simulink model "isitici"  (R2026b)
settings: Solver=VariableStepAuto  StopTime=1200  MaxStep=0.1
values from neighbouring files (symbols this model uses):
  Chx = 10000    [init_params.m]
  cpw = 4186    [init_params.m]    (also in test_ch_low.m)
  Crad = 100000    [init_params.m]
  Croom = 2e6    (= 2000000)    [init_params.m]
  dTmax = 30    [init_params.m]
  etanom = 0.975    [init_params.m]
  etax = [30 55 80]    [init_params.m]
  etay = [1.02 0.975 0.975]    [init_params.m]
  hcmode = 1    [init_params.m]    (also in test_hc.m = 2; test_room.m = 2)
  hcx = [-15 -5 5 15 20]    [init_params.m]
  hcy = [75 62 49 36 30]    [init_params.m]    (also in test_hc.m = hcy_backup)
  Kir = 0.002    [init_params.m]
  Kpr = 10    [init_params.m]
  Krad = 35.2    [init_params.m]
  Ktr = 0.5    [init_params.m]
  mdot = 0.25    [init_params.m]
  nmax = 3    [init_params.m]
  nrad = 1.3    [init_params.m]
  Qgasmax = 24600    [init_params.m]
  Qmax = 24000    [init_params.m]
  Qmin = Qmax/turndown    (= 2400)    [init_params.m]
  Tamb = Troomset    (= 21)    [test_room.m]
  tauntc = 5    [init_params.m]
  tflame = 1    [init_params.m]
  tflamefail = 300    [export_ref.m]    (also in init_params.m = 1000000000; testseq.m)
  Tflowmax = 75    [init_params.m]
  Tflowmin = 30    [init_params.m]
  tignsafety = 3    [init_params.m]
  Tlimit = 90    [init_params.m]
  tminoff = 60    [init_params.m]
  tminon = 100;',   1200    [export_ref.m]    (also in init_params.m = 30; testseq.m = 100)
  Toutamp = 0    [init_params.m]    (also in test_room.m = 4)
  Toutdoor = -25    [test_hc.m]    (also in test_room.m = 5)
  tpostpurge = 10    [init_params.m]
  tprepurge = 5    [init_params.m]
  Troomset = 21    [init_params.m]    (also in test_room.m)
  trst = 330;',             400    [export_ref.m]    (also in init_params.m = 1000000000; testseq.m = 330)
  Tsch = 0.1    [init_params.m]
  Tsmax = 40;',                             100    [export_ref.m]    (also in init_params.m = 130; testseq.m = 40)
  Tsmin = -20    [init_params.m]
  Tsr = 1    [init_params.m]
  Tstb = 50;',                              120    [export_ref.m]    (also in init_params.m = 95; testseq.m = 50)
  tstep = 200    [init_params.m]    (also in test_ch_basic.m; test_ch_step.m = 400)
  UAh = 190    [init_params.m]    (also in test_room.m = 190*f)
libraries: slpidlib x1
settings Model: Creator=Ogun Serif  LastModifiedBy=ogunserifonargan

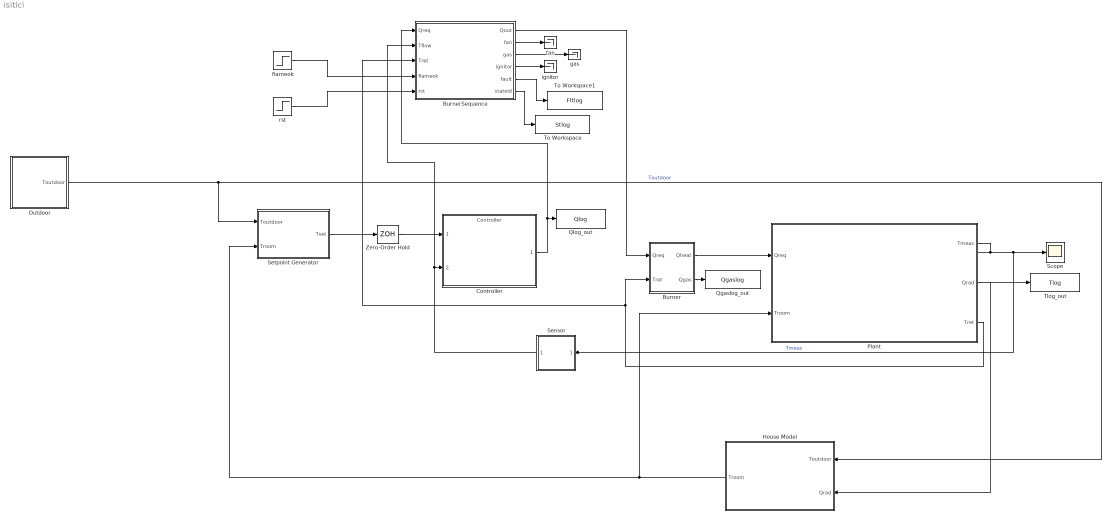
== system isitici ==
  Burner : Subsystem
  BurnerSequence : Stateflow chart  TreatAsAtomicUnit=on
  Controller : ModelReference  ModelNameDialog=Controller  SimulationMode=Normal  ModelReferenceVersion=1.11
  House Model : Subsystem
  Outdoor : Subsystem
  Plant : Subsystem
  Qgaslog_out : ToWorkspace  VariableName=Qgaslog  SaveFormat=Timeseries  SampleTime=-1
  Qlog_out : ToWorkspace  VariableName=Qlog  SaveFormat=Timeseries  SampleTime=0.1
  Scope : Scope
      settings: ActiveDisplayYMinimum=43.32281343157301  ActiveDisplayYMaximum=61.925815623975161
  Sensor : Subsystem
  Setpoint Generator : Subsystem
  Tlog_out : ToWorkspace  VariableName=Tlog  SaveFormat=Timeseries  SampleTime=0.1
  To Workspace : ToWorkspace  VariableName=Stlog  SaveFormat=Timeseries  SampleTime=0.1
  To Workspace1 : ToWorkspace  VariableName=Fltlog  SaveFormat=Timeseries  SampleTime=0.1
  Zero-Order Hold : ZeroOrderHold  SampleTime=Tsch
  fan : Terminator
  flameok : Step  Time=tflamefail  InitialValue=1  FinalValue=0  SampleTime=0
  gas : Terminator
  ignitor : Terminator
  rst : Step  Time=trst  SampleTime=0
  wires:
  Zero-Order Hold/1 -> Controller/1
  Plant/1(Tmeas) -> Sensor/1(Tmeas), Scope/1, Tlog_out/1  "Tmeas"
  Controller/1 -> BurnerSequence/1(Qreq), Qlog_out/1
  Outdoor/1(Toutdoor) -> Setpoint Generator/1(Toutdoor), House Model/1(Toutdoor)  "Toutdoor"
  House Model/1(Troom) -> Setpoint Generator/2(Troom), Plant/2(Troom)
  Setpoint Generator/1(Tset) -> Zero-Order Hold/1
  Plant/2(Qrad) -> House Model/2(Qrad)
  Sensor/1(Tsens) -> BurnerSequence/2(Tflow), Controller/2
  Burner/1(Qheat) -> Plant/1(Qreq)
  Plant/3(Tret) -> BurnerSequence/3(Tret), Burner/2(Tret)
  Burner/2(Qgas) -> Qgaslog_out/1
  BurnerSequence/1(Qout) -> Burner/1(Qreq)
  flameok/1 -> BurnerSequence/4(flameok)
  rst/1 -> BurnerSequence/5(rst)
  BurnerSequence/6(stateid) -> To Workspace/1
  BurnerSequence/5(fault) -> To Workspace1/1
  BurnerSequence/2(fan) -> fan/1
  BurnerSequence/3(gas) -> gas/1
  BurnerSequence/4(ignitor) -> ignitor/1

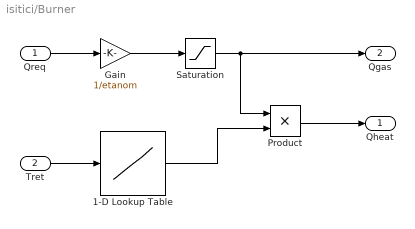
== system isitici/Burner ==
  Qreq : Inport
  Tret : Inport  Port=2
  1-D Lookup Table : Lookup_n-D  NumberOfTableDimensions=1  BreakpointsForDimension1=etax  Table=etay  ExtrapMethod=Clip  InternalRulePriority=Speed  RndMeth=Simplest
  Gain : Gain  Gain=1/etanom
  Product : Product
  Saturation : Saturate  UpperLimit=Qgasmax  LowerLimit=0
  Qheat : Outport
  Qgas : Outport  Port=2
  wires:
  Qreq/1 -> Gain/1
  Gain/1 -> Saturation/1
  Saturation/1 -> Qgas/1, Product/1
  Product/1 -> Qheat/1
  Tret/1 -> 1-D Lookup Table/1
  1-D Lookup Table/1 -> Product/2

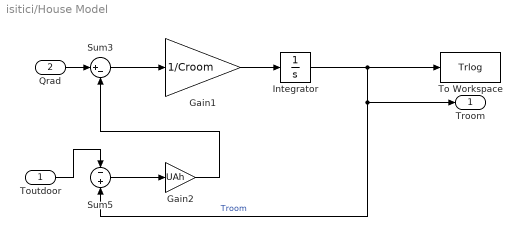
== system isitici/House Model ==
  Toutdoor : Inport
  Qrad : Inport  Port=2
  Gain1 : Gain  Gain=1/Croom
  Gain2 : Gain  Gain=UAh
  Integrator : Integrator  InitialCondition=Tamb
  Sum3 : Sum  Inputs=|+-
  Sum5 : Sum  Inputs=-+
  To Workspace : ToWorkspace  VariableName=Trlog  SaveFormat=Timeseries  SampleTime=10
  Troom : Outport
  wires:
  Integrator/1 -> To Workspace/1, Sum5/2, Troom/1  "Troom"
  Gain1/1 -> Integrator/1
  Qrad/1 -> Sum3/1
  Sum5/1 -> Gain2/1
  Sum3/1 -> Gain1/1
  Gain2/1 -> Sum3/2
  Toutdoor/1 -> Sum5/1

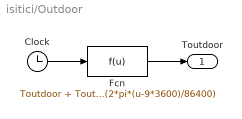
== system isitici/Outdoor ==
  Clock : Clock
  Fcn : Fcn  Expr=Toutdoor + Toutamp*sin(2*pi*(u-9*3600)/86400)
  Toutdoor : Outport
  wires:
  Fcn/1 -> Toutdoor/1
  Clock/1 -> Fcn/1

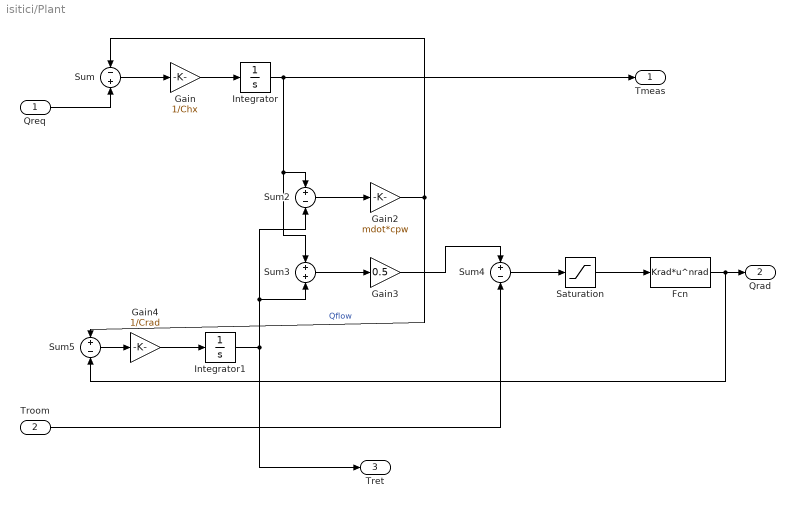
== system isitici/Plant ==
  Qreq : Inport
  Troom : Inport  Port=2
  Fcn : Fcn  Expr=Krad*u^nrad
  Gain : Gain  Gain=1/Chx
  Gain2 : Gain  Gain=mdot*cpw
  Gain3 : Gain  Gain=0.5
  Gain4 : Gain  Gain=1/Crad
  Integrator : Integrator  InitialCondition=Tamb
  Integrator1 : Integrator  InitialCondition=Tamb
  Saturation : Saturate  UpperLimit=inf  LowerLimit=0
  Sum : Sum  Inputs=-|+
  Sum2 : Sum  Inputs=+|-
  Sum3 : Sum  Inputs=+|+
  Sum4 : Sum  Inputs=+|-
  Sum5 : Sum  Inputs=+|-
  Tmeas : Outport
  Qrad : Outport  Port=2
  Tret : Outport  Port=3
  wires:
  Integrator/1 -> Sum2/1, Sum3/1, Tmeas/1
  Gain/1 -> Integrator/1
  Sum/1 -> Gain/1
  Qreq/1 -> Sum/2
  Sum2/1 -> Gain2/1
  Gain2/1 -> Sum5/1, Sum/1  "Qflow"
  Sum3/1 -> Gain3/1
  Gain3/1 -> Sum4/1
  Sum4/1 -> Saturation/1
  Saturation/1 -> Fcn/1
  Fcn/1 -> Sum5/2, Qrad/1
  Sum5/1 -> Gain4/1
  Gain4/1 -> Integrator1/1
  Integrator1/1 -> Tret/1, Sum3/2, Sum2/2
  Troom/1 -> Sum4/2

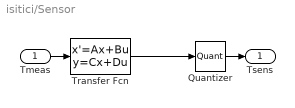
== system isitici/Sensor ==
  Tmeas : Inport
  Quantizer : Quantizer  QuantizationInterval=qntc
  Transfer Fcn : StateSpace  A=-1/tauntc  B=1/tauntc  D=0  InitialCondition=Tamb
  Tsens : Outport
  wires:
  Transfer Fcn/1 -> Quantizer/1
  Tmeas/1 -> Transfer Fcn/1
  Quantizer/1 -> Tsens/1

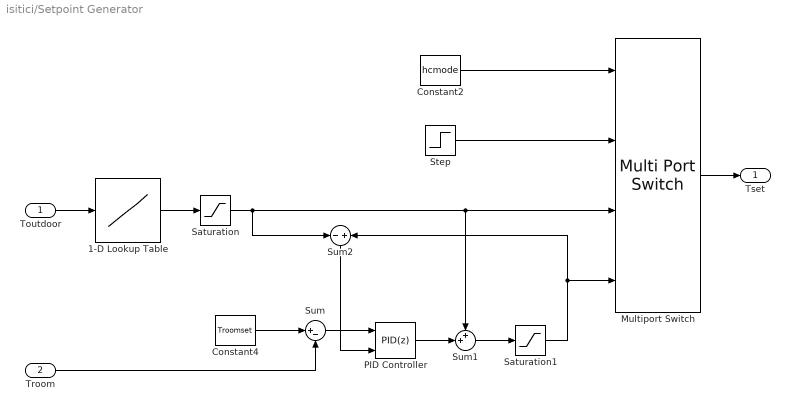
== system isitici/Setpoint Generator ==
  Toutdoor : Inport
  Troom : Inport  Port=2
  1-D Lookup Table : Lookup_n-D  NumberOfTableDimensions=1  BreakpointsForDimension1=hcx  Table=hcy  InternalRulePriority=Speed  RndMeth=Simplest
  Constant2 : Constant  Value=hcmode
  Constant4 : Constant  Value=Troomset
  Multiport Switch : MultiPortSwitch  SaturateOnIntegerOverflow=off  InputSameDT=off
  PID Controller : slpidlib/PID Controller  Controller=PID  Form=Parallel  TimeDomain=Discrete-time  UseExternalTs=off  SampleTime=Tsr  IntegratorMethod=Forward Euler  FilterMethod=Forward Euler  ControllerParametersSource=internal  P=Kpr  I=Kir  UseKiTs=off  D=0  UseExternalDerivativeSource=off  N=100  UseFilter=on  TunerSelectOption=Transfer Function Based (PID Tuner App)  InitialConditionSource=internal  InitialConditionForIntegrator=0  InitialConditionForFilter=0  DifferentiatorICPrevScaledInput=0  ExternalReset=none  TrackingMode=on  Kt=Ktr  LimitOutput=off  SatLimitsSource=internal  UpperSaturationLimit=inf  LowerSaturationLimit=-inf  LinearizeAsGain=on  AntiWindupMode=none  Kb=1  LimitIntegrator=off  UpperIntegratorSaturationLimit=inf  LowerIntegratorSaturationLimit=-inf  POutMin=[]  POutMax=[]  IOutMin=[]  IOutMax=[]  DOutMin=[]  DOutMax=[]  NOutMin=[]  NOutMax=[]  SumOutMin=[]  SumOutMax=[]  SaturationOutMin=[]  SaturationOutMax=[]  PParamMin=[]  PParamMax=[]  IParamMin=[]  IParamMax=[]  DParamMin=[]  DParamMax=[]  NParamMin=[]  NParamMax=[]  KbParamMin=[]  KbParamMax=[]  KtParamMin=[]  KtParamMax=[]  KbOutMin=[]  KbOutMax=[]  KtOutMin=[]  KtOutMax=[]  IntegratorOutMin=[]  IntegratorOutMax=[]  FilterOutMin=[]  FilterOutMax=[]  SumI1OutMin=[]  SumI1OutMax=[]  SumI2OutMin=[]  SumI2OutMax=[]  SumI3OutMin=[]  SumI3OutMax=[]  SumI4OutMin=[]  SumI4OutMax=[]  SumDOutMin=[]  SumDOutMax=[]  DifferentiatorOutMin=[]  DifferentiatorOutMax=[]  FilterDiffOutCoefMin=[]  FilterDiffOutCoefMax=[]  ReciprocalOutMin=[]  ReciprocalOutMax=[]  SumDenOutMin=[]  SumDenOutMax=[]  SumNumOutMin=[]  SumNumOutMax=[]  DivideOutMin=[]  DivideOutMax=[]  UdiffTsProdOutMin=[]  UdiffTsProdOutMax=[]  NTsProdOutMin=[]  NTsProdOutMax=[]  UintegralTsProdOutMin=[]  UintegralTsProdOutMax=[]  UngainTsProdOutMin=[]  UngainTsProdOutMax=[]  ClampingZeroOutDataTypeStr=Inherit: Inherit via back propagation  ClampingZeroOutMin=[]  ClampingZeroOutMax=[]  FilterDenConstantOutDataTypeStr=Inherit: Inherit via back propagation  FilterDenConstantOutMin=[]  FilterDenConstantOutMax=[]  PCopyOutDataTypeStr=Inherit: Inherit via back propagation  PCopyOutMin=[]  PCopyOutMax=[]  NCopyOutDataTypeStr=Inherit: Inherit via back propagation  NCopyOutMin=[]  NCopyOutMax=[]  IntegratorContinuousStateAttributes=''  IntegratorStateMustResolveToSignalObject=off  IntegratorRTWStateStorageClass=Auto  FilterContinuousStateAttributes=''  FilterStateMustResolveToSignalObject=off  FilterRTWStateStorageClass=Auto  ParallelPVariant=InternalParameters  IdealPVariant=Disabled  IVariant=InternalParameters  DVariant=InternalParameters  IntegratorVariant=Discrete  SatVariant=Disabled  AWVariant=Passthrough  PCopyVariant=Disabled  TRVariant=Enabled  FdbkBlocksVariant=Forward  IdealPFdbkVariant=Disabled  SatFdbkVariant=Disabled  DerivativeFilterVariant=ForwardEulerFilter  NVariant=InternalParameters  NCopyVariant=Disabled  FilterICVariant=InternalICsFilter  IntegratorICVariant=InternalICs  ExternalResetVariant=Disabled  TRSumVariant=TrackingMode  SumFdbkVariant=Disabled  SumVariant=Sum_PID  TsampFilterVariant=InternalTs  TsampNgainVariant=Passthrough  TsampIntegralVariant=Disabled_SignalSpec  ExternalSaturationOutDataTypeStr=Inherit: Same as second input  DerivativeSourceVariant=ErrorSignal  PreIntVariant=InternalPreInt
  Saturation : Saturate  UpperLimit=Tflowmax  LowerLimit=Tflowmin
  Saturation1 : Saturate  UpperLimit=Tflowmax  LowerLimit=Tflowmin
  Step : Step  Time=tstep  InitialValue=tsetinit  FinalValue=tsetfinal  SampleTime=0
  Sum : Sum  Inputs=|+-
  Sum1 : Sum  Inputs=++|
  Sum2 : Sum  Inputs=-+
  Tset : Outport
  wires:
  Multiport Switch/1 -> Tset/1
  Saturation1/1 -> Multiport Switch/4, Sum2/2
  Constant2/1 -> Multiport Switch/1
  Sum1/1 -> Saturation1/1
  Sum/1 -> PID Controller/1
  Sum2/1 -> PID Controller/2
  Step/1 -> Multiport Switch/2
  PID Controller/1 -> Sum1/2
  Troom/1 -> Sum/2
  Constant4/1 -> Sum/1
  Saturation/1 -> Sum1/1, Multiport Switch/3, Sum2/1
  1-D Lookup Table/1 -> Saturation/1
  Toutdoor/1 -> 1-D Lookup Table/1

== stateflow chart isitici/BurnerSequence ==
  settings: updateMethod=DISCRETE  sampleTime=Tsch
  state Operation
    entry:
    fault = 0;
    state Idle
      entry:
      fan = 0; gas = 0; ignitor = 0; Qout = 0; stateid = 0;
    state PrePurge
      entry:
      fan = 1; gas = 0; ignitor = 0; Qout = 0; stateid = 1;
    state Ignition
      entry:
      gas = 1; ignitor = 1; Qout = 0; stateid = 2; ntry = ntry + 1;
    state Run
      entry:
      ignitor = 0; stateid = 3;
      during:
      Qout = Qreq;
      if Tflow > Tlimit
      Qout = Qreq*(Tstb - Tflow)/(Tstb - Tlimit);
      end
      if Tflow - Tret > dTmax
      Qout = Qmin;
      end
      Qout = min(max(Qout, Qmin), Qmax);
    state PostPurge
      entry:
      gas = 0; ignitor = 0; Qout = 0; fan = 1; stateid = 4;
    state Wait
      entry:
      fan = 0; stateid = 5;
    (default) -> Idle
    Wait -> Idle : [after(tminoff,sec)]
    Idle -> PrePurge : [Qreq > 0]{ntry = 0;}
    Ignition -> PrePurge [order 2] : [flameok <= 0 && after(tignsafety,sec) && ntry < nmax]
    PrePurge -> Ignition : [after(tprepurge,sec)]
    Ignition -> Run [order 1] : [flameok > 0 && after(tflame,sec)]
    Run -> PostPurge [order 1] : [Qreq <= 0 && after(tminon,sec)]
    PostPurge -> Wait : [after(tpostpurge,sec)]
  state Lockout
    entry:
    gas = 0; fan = 0; ignitor = 0; Qout = 0; stateid = 6;
  note: [flameok <= 0 && after(tignsafety,sec) && ntry >= nmax]{fault = 3;}
  Lockout -> Operation : [rst > 0]
  Ignition -> Lockout [order 3] : [flameok <= 0 && after(tignsafety,sec) && ntry >= nmax]{fault = 3;}
  Operation -> Lockout [order 1] : [Tflow > Tstb && Tflow <= Tsmax]{fault = 1;}
  Run -> Lockout [order 2] : [flameok <= 0]{fault = 4;}
  Operation -> Lockout [order 2] : [Tflow < Tsmin || Tflow > Tsmax]{fault = 2;}
  (default) -> Operation
  data: Qreq input; Tflow input; Tret input; flameok input; rst input; Qout output; fan output; gas output; ignitor output; fault output; stateid output; ntry local; tprepurge parameter; tflame parameter; tignsafety parameter; nmax parameter; tpostpurge parameter; tminoff parameter; tminon parameter; Tstb parameter; Tlimit parameter; dTmax parameter; Tsmin parameter; Tsmax parameter; Qmin parameter; Qmax parameter
